simulink model "Crosswalk_Control"  (R2026a)
settings: Solver=VariableStepAuto
settings Model: Creator=wyatt  LastModifiedBy=wyatt

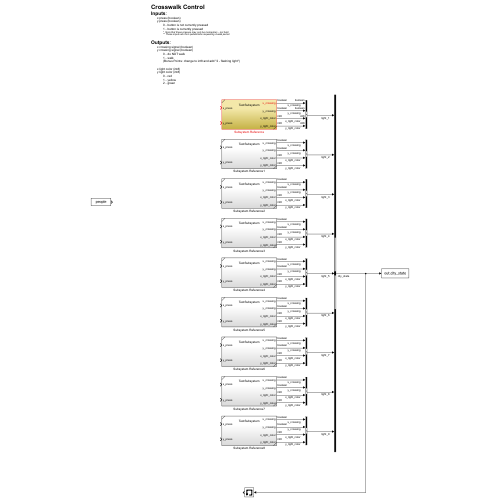
[thumbnail: Simulink's stored preview of the top-level diagram]
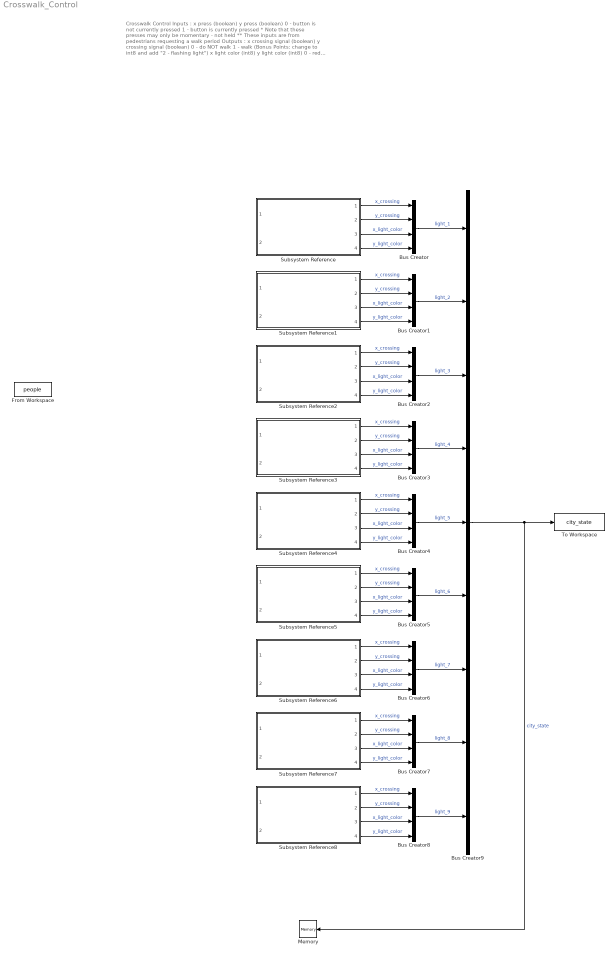
== system Crosswalk_Control ==
  note: Crosswalk Control
      | Inputs :
      | x press (boolean)
      | y press (boolean)
      | 0 - button is not currently pressed
      | 1 - button is currently pressed
      | * Note that these presses may only be momentary - not held
      | ** These inputs are from pedestrians requesting a walk period
      |
      | Outputs :
      | x crossing signal (boolean)
      | y crossing signal (boolean)
      | 0 - do NOT walk
      | 1 - walk
      | (Bonus Points: change to int8 and add "2 - flashing light")
      |
      | x light color (int8)
      | y light color (int8)
      | 0 - red
      | 1 - yellow
      | 2 - green
  Bus Creator{,1..8} (9 alike) : BusCreator  Inputs=4
  Bus Creator9 : BusCreator  Inputs=9
  From Workspace : FromWorkspace  VariableName=people  OutputAfterFinalValue=Holding final value
  Memory : Memory
  Subsystem Reference{,1..8} (9 alike) : Subsystem  ReferencedSubsystem=TestSubsystem
  To Workspace : ToWorkspace  VariableName=city_state  SaveFormat=Structure With Time  SampleTime=-1
  wires:
  Subsystem Reference/1 -> Bus Creator/1  "x_crossing"
  Subsystem Reference/2 -> Bus Creator/2  "y_crossing"
  Subsystem Reference/3 -> Bus Creator/3  "x_light_color"
  Subsystem Reference/4 -> Bus Creator/4  "y_light_color"
  Bus Creator/1 -> Bus Creator9/1  "light_1"
  Subsystem Reference1/1 -> Bus Creator1/1  "x_crossing"
  Subsystem Reference1/2 -> Bus Creator1/2  "y_crossing"
  Bus Creator1/1 -> Bus Creator9/2  "light_2"
  Subsystem Reference1/3 -> Bus Creator1/3  "x_light_color"
  Subsystem Reference1/4 -> Bus Creator1/4  "y_light_color"
  Subsystem Reference2/1 -> Bus Creator2/1  "x_crossing"
  Subsystem Reference3/3 -> Bus Creator3/3  "x_light_color"
  Subsystem Reference3/4 -> Bus Creator3/4  "y_light_color"
  Subsystem Reference3/2 -> Bus Creator3/2  "y_crossing"
  Subsystem Reference2/2 -> Bus Creator2/2  "y_crossing"
  Bus Creator3/1 -> Bus Creator9/4  "light_4"
  Bus Creator2/1 -> Bus Creator9/3  "light_3"
  Subsystem Reference3/1 -> Bus Creator3/1  "x_crossing"
  Subsystem Reference2/3 -> Bus Creator2/3  "x_light_color"
  Subsystem Reference2/4 -> Bus Creator2/4  "y_light_color"
  Subsystem Reference4/1 -> Bus Creator4/1  "x_crossing"
  Subsystem Reference5/3 -> Bus Creator5/3  "x_light_color"
  Subsystem Reference5/4 -> Bus Creator5/4  "y_light_color"
  Subsystem Reference5/2 -> Bus Creator5/2  "y_crossing"
  Subsystem Reference4/2 -> Bus Creator4/2  "y_crossing"
  Bus Creator5/1 -> Bus Creator9/6  "light_6"
  Bus Creator4/1 -> Bus Creator9/5  "light_5"
  Subsystem Reference5/1 -> Bus Creator5/1  "x_crossing"
  Subsystem Reference4/3 -> Bus Creator4/3  "x_light_color"
  Subsystem Reference4/4 -> Bus Creator4/4  "y_light_color"
  Subsystem Reference6/1 -> Bus Creator6/1  "x_crossing"
  Subsystem Reference7/3 -> Bus Creator7/3  "x_light_color"
  Subsystem Reference7/4 -> Bus Creator7/4  "y_light_color"
  Subsystem Reference7/2 -> Bus Creator7/2  "y_crossing"
  Subsystem Reference6/2 -> Bus Creator6/2  "y_crossing"
  Bus Creator7/1 -> Bus Creator9/8  "light_8"
  Bus Creator6/1 -> Bus Creator9/7  "light_7"
  Subsystem Reference7/1 -> Bus Creator7/1  "x_crossing"
  Subsystem Reference6/3 -> Bus Creator6/3  "x_light_color"
  Subsystem Reference6/4 -> Bus Creator6/4  "y_light_color"
  Subsystem Reference8/1 -> Bus Creator8/1  "x_crossing"
  Subsystem Reference8/2 -> Bus Creator8/2  "y_crossing"
  Bus Creator8/1 -> Bus Creator9/9  "light_9"
  Subsystem Reference8/3 -> Bus Creator8/3  "x_light_color"
  Subsystem Reference8/4 -> Bus Creator8/4  "y_light_color"
  Bus Creator9/1 -> To Workspace/1, Memory/1  "city_state"
